simulink model "exp6"  (R2025a)
settings: Solver=VariableStepAuto  StartTime=0.0  StopTime=10.0  RelTol=1e-3
libraries: spsSeriesRLCBranchLib x12, spsGroundLib x2, spsThreePhaseVIMeasurementLib x2, spsThreePhaseSourceLib x2
settings Model: Creator=USER  LastModifiedBy=USER

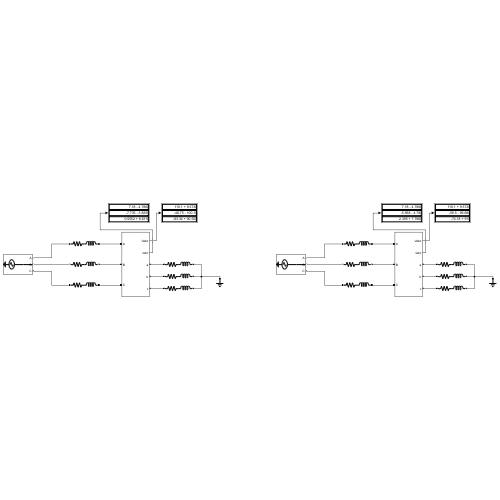
[thumbnail: Simulink's stored preview of the top-level diagram]
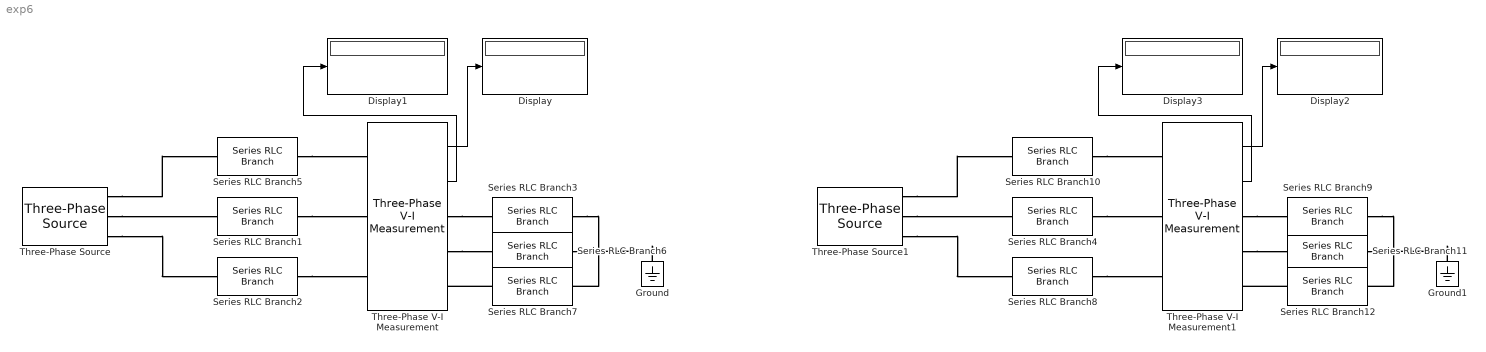
== system exp6 ==
  Display{,1..3} (4 alike) : Display
  Ground : spsGroundLib/Ground  LConnTagsString=a
  Ground1 : spsGroundLib/Ground  LConnTagsString=a
  Series RLC Branch{1..2,4..5,8,10} (6 alike) : spsSeriesRLCBranchLib/Series RLC Branch  LConnTagsString=__new0  RConnTagsString=__new0  BranchType=RL  Resistance=5  Inductance=5.305e-3  SetiL0=off  InitialCurrent=0  Capacitance=1e-6  Setx0=off  InitialVoltage=0  Measurements=None
  Series RLC Branch11 : spsSeriesRLCBranchLib/Series RLC Branch  LConnTagsString=__new0  RConnTagsString=__new0  BranchType=RL  Resistance=15  Inductance=13.33e-3  SetiL0=off  InitialCurrent=0  Capacitance=1e-6  Setx0=off  InitialVoltage=0  Measurements=None
  Series RLC Branch12 : spsSeriesRLCBranchLib/Series RLC Branch  LConnTagsString=__new0  RConnTagsString=__new0  BranchType=RL  Resistance=8  Inductance=31.8e-3  SetiL0=off  InitialCurrent=0  Capacitance=1e-6  Setx0=off  InitialVoltage=0  Measurements=None
  Series RLC Branch{3,6..7,9} (4 alike) : spsSeriesRLCBranchLib/Series RLC Branch  LConnTagsString=__new0  RConnTagsString=__new0  BranchType=RL  Resistance=10  Inductance=21.22e-3  SetiL0=off  InitialCurrent=0  Capacitance=1e-6  Setx0=off  InitialVoltage=0  Measurements=None
  Three-Phase V-I Measurement : spsThreePhaseVIMeasurementLib/Three-Phase V-I Measurement  VoltageMeasurement=phase-to-ground  SetLabelV=off  LabelV=Vabc  Vpu=off  VpuLL=off  CurrentMeasurement=yes  SetLabelI=off  LabelI=Iabc  Ipu=off  Pbase=100e6  Vbase=500e3  OutputType=Complex  PhasorSimulation=on  PSBequivalent=0
  Three-Phase V-I Measurement1 : spsThreePhaseVIMeasurementLib/Three-Phase V-I Measurement  VoltageMeasurement=phase-to-ground  SetLabelV=off  LabelV=Vabc  Vpu=off  VpuLL=off  CurrentMeasurement=yes  SetLabelI=off  LabelI=Iabc  Ipu=off  Pbase=100e6  Vbase=500e3  OutputType=Complex  PhasorSimulation=on  PSBequivalent=0
  Three-Phase Source : spsThreePhaseSourceLib/Three-Phase Source  InternalConnection=Yg  VoltagePhases=off  Voltage=190.525  PhaseAngle=0  Voltage_phases=[25e3 25e3 25e3]/sqrt(3)  PhaseAngles_phases=[0 -120 +120]  Frequency=60  NonIdealSource=off  SpecifyImpedance=off  Resistance=0.8929  Inductance=16.58e-3  ShortCircuitLevel=100e6  BaseVoltage=25e3  XRratio=7  BusType=swing  Pref=10e3  Qref=0  Prefabc=[10e3, 10e3, 10e3]  Qrefabc=[0, 0, 0]  Qmin=-inf  Qmax=inf
  Three-Phase Source1 : spsThreePhaseSourceLib/Three-Phase Source  InternalConnection=Yg  VoltagePhases=off  Voltage=190.525  PhaseAngle=0  Voltage_phases=[25e3 25e3 25e3]/sqrt(3)  PhaseAngles_phases=[0 -120 +120]  Frequency=60  NonIdealSource=off  SpecifyImpedance=off  Resistance=0.8929  Inductance=16.58e-3  ShortCircuitLevel=100e6  BaseVoltage=25e3  XRratio=7  BusType=swing  Pref=10e3  Qref=0  Prefabc=[10e3, 10e3, 10e3]  Qrefabc=[0, 0, 0]  Qmin=-inf  Qmax=inf
  wires:
  Three-Phase V-I Measurement/1 -> Display/1
  Three-Phase V-I Measurement/2 -> Display1/1
  Three-Phase V-I Measurement1/2 -> Display3/1
  Three-Phase V-I Measurement1/1 -> Display2/1
  connections:
  Three-Phase Source/RConn2 -- Series RLC Branch1/LConn1
  Series RLC Branch1/RConn1 -- Three-Phase V-I Measurement/LConn2
  Series RLC Branch5/RConn1 -- Three-Phase V-I Measurement/LConn1
  Series RLC Branch2/RConn1 -- Three-Phase V-I Measurement/LConn3
  Three-Phase Source/RConn1 -- Series RLC Branch5/LConn1
  Three-Phase Source/RConn3 -- Series RLC Branch2/LConn1
  Series RLC Branch7/LConn1 -- Three-Phase V-I Measurement/RConn3
  Three-Phase V-I Measurement/RConn2 -- Series RLC Branch6/LConn1
  Three-Phase V-I Measurement/RConn1 -- Series RLC Branch3/LConn1
  Series RLC Branch3/RConn1 -- Ground/LConn1 -- Series RLC Branch6/RConn1 -- Series RLC Branch7/RConn1
  Series RLC Branch9/RConn1 -- Ground1/LConn1 -- Series RLC Branch11/RConn1 -- Series RLC Branch12/RConn1
  Three-Phase Source1/RConn3 -- Series RLC Branch8/LConn1
  Series RLC Branch12/LConn1 -- Three-Phase V-I Measurement1/RConn3
  Series RLC Branch4/RConn1 -- Three-Phase V-I Measurement1/LConn2
  Three-Phase Source1/RConn1 -- Series RLC Branch10/LConn1
  Series RLC Branch8/RConn1 -- Three-Phase V-I Measurement1/LConn3
  Three-Phase Source1/RConn2 -- Series RLC Branch4/LConn1
  Three-Phase V-I Measurement1/RConn2 -- Series RLC Branch11/LConn1
  Three-Phase V-I Measurement1/RConn1 -- Series RLC Branch9/LConn1
  Series RLC Branch10/RConn1 -- Three-Phase V-I Measurement1/LConn1
